simulink model "ElevatorRegen_OptB_L2"  (R2024b)
settings: Solver=FixedStepDiscrete  StartTime=0.0  StopTime=25  FixedStep=Ts_power  RelTol=1e-3
values from neighbouring files (symbols this model uses):
  Cdc = 2.2e-3    (= 0.0022)    [params_elevator.m]
  f_g = 50    [params_elevator.m]
  L_acd = 0.5e-3    (= 0.0005)    [params_elevator.m]
  L_f = L1 + L2    [params_elevator.m]
  Lg = XR*Rg/w_g    [params_elevator.m]
  R_acd = 5e-3    (= 0.005)    [params_elevator.m]
  R_f = 0.005*Z_B    (= 0.0666666666667)    [params_elevator.m]
  Rb_B = Vchop_on^2/P_DC_regen_peak    (= 48.4015424137)    [params_elevator.m]
  Rg = Zg/sqrt(1+XR^2)    [params_elevator.m]
  SIGNE_ISRC = +1    (= 1)    [build_optionB_L2.m]
  Ts_ctrl = 1/fsw    (= 0.0001)    [params_elevator.m]
  Ts_power = Ts_ctrl/2    (= 5e-05)    [params_elevator.m]
  V_LL = 400    [params_elevator.m]
  Vchop_off = 740    [params_elevator.m]
  Vchop_on = 760    [params_elevator.m]
libraries: spsThreePhaseSeriesRLCBranchLib x3, spsControlledVoltageSourceLib x3, spsSeriesRLCBranchLib x2, spsControlledCurrentSourceLib x2, spsThreePhaseVIMeasurementLib x2, spsIdealSwitchLib x1, spsVoltageMeasurementLib x1, spsUniversalBridgeLib x1, spsThreePhaseSourceLib x1, spspowerguiLib x1
settings Model: Creator=Med Amine  LastModifiedBy=Med Amine

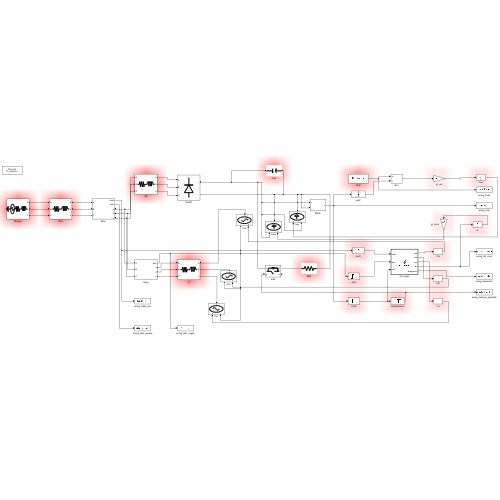
[thumbnail: Simulink's stored preview of the top-level diagram]
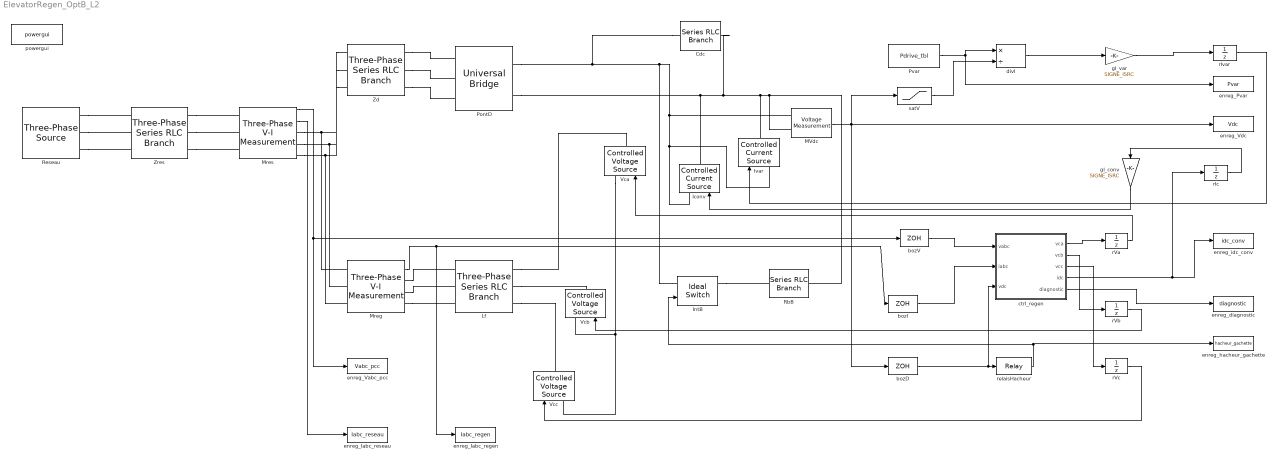
== system ElevatorRegen_OptB_L2 ==
  Cdc : spsSeriesRLCBranchLib/Series RLC Branch  LConnTagsString=__new0  RConnTagsString=__new0  BranchType=C  Resistance=1  Inductance=1e-3  SetiL0=on  InitialCurrent=0  Capacitance=Cdc  Setx0=off  InitialVoltage=Vdc0  Measurements=None
  Iconv : spsControlledCurrentSourceLib/Controlled Current Source  Initialize=on  Source_Type=AC  Amplitude=0  Phase=0  Frequency=0  Measurements=None
  IntB : spsIdealSwitchLib/Ideal Switch  Ron=1e-3  Lon=0  IC=0  Rs=1e6  Cs=inf  Measurements=on
  Ivar : spsControlledCurrentSourceLib/Controlled Current Source  Initialize=on  Source_Type=AC  Amplitude=0  Phase=0  Frequency=0  Measurements=None
  Lf : spsThreePhaseSeriesRLCBranchLib/Three-Phase Series RLC Branch  LConnTagsString=A|B|C  RConnTagsString=A|B|C  BranchType=RL  Resistance=R_f  Inductance=L_f  Capacitance=1e-6  Measurements=None
  MVdc : spsVoltageMeasurementLib/Voltage Measurement  PhasorSimulation=off  OutputType=Complex  PSBequivalent=0
  Mreg : spsThreePhaseVIMeasurementLib/Three-Phase V-I Measurement  VoltageMeasurement=no  SetLabelV=off  LabelV=Vabc  Vpu=off  VpuLL=off  CurrentMeasurement=yes  SetLabelI=off  LabelI=Iabc  Ipu=off  Pbase=100e6  Vbase=500e3  OutputType=Complex  PhasorSimulation=off  PSBequivalent=0
  Mres : spsThreePhaseVIMeasurementLib/Three-Phase V-I Measurement  VoltageMeasurement=phase-to-ground  SetLabelV=off  LabelV=Vabc  Vpu=off  VpuLL=off  CurrentMeasurement=yes  SetLabelI=off  LabelI=Iabc  Ipu=off  Pbase=100e6  Vbase=500e3  OutputType=Complex  PhasorSimulation=off  PSBequivalent=0
  PontD : spsUniversalBridgeLib/Universal Bridge  Arms=3  SnubberResistance=1e5  SnubberCapacitance=inf  Device=Diodes  Ron=1e-3  Lon=0  ForwardVoltages="[  0  0  ]"  ForwardVoltage=0.8  GTOparameters=[ 10e-6 , 20e-6 ]  IGBTparameters=[ 1e-6 , 2e-6 ]  Measurements=None  Measurements_2=None  converterType=Rectifier
  Pvar : FromWorkspace  VariableName=Pdrive_tbl  OutputAfterFinalValue=Setting to zero
  RbB : spsSeriesRLCBranchLib/Series RLC Branch  LConnTagsString=__new0  RConnTagsString=__new0  BranchType=R  Resistance=Rb_B  Inductance=1e-3  SetiL0=off  InitialCurrent=0  Capacitance=1e-6  Setx0=off  InitialVoltage=0  Measurements=None
  Reseau : spsThreePhaseSourceLib/Three-Phase Source  InternalConnection=Yg  VoltagePhases=off  Voltage=V_LL  PhaseAngle=0  Voltage_phases=[25e3 25e3 25e3]/sqrt(3)  PhaseAngles_phases=[0 -120 +120]  Frequency=f_g  NonIdealSource=on  SpecifyImpedance=off  Resistance=0.8929  Inductance=16.58e-3  ShortCircuitLevel=100e6  BaseVoltage=25e3  XRratio=7  BusType=swing  Pref=10e3  Qref=0  Prefabc=[10e3, 10e3, 10e3]  Qrefabc=[0, 0, 0]  Qmin=-inf  Qmax=inf
  Vca : spsControlledVoltageSourceLib/Controlled Voltage Source  Initialize=on  Source_Type=AC  Amplitude=0  Phase=0  Frequency=0  Measurements=None
  Vcb : spsControlledVoltageSourceLib/Controlled Voltage Source  Initialize=on  Source_Type=AC  Amplitude=0  Phase=0  Frequency=0  Measurements=None
  Vcc : spsControlledVoltageSourceLib/Controlled Voltage Source  Initialize=on  Source_Type=AC  Amplitude=0  Phase=0  Frequency=0  Measurements=None
  Zd : spsThreePhaseSeriesRLCBranchLib/Three-Phase Series RLC Branch  LConnTagsString=A|B|C  RConnTagsString=A|B|C  BranchType=RL  Resistance=R_acd  Inductance=L_acd  Capacitance=1e-6  Measurements=None
  Zres : spsThreePhaseSeriesRLCBranchLib/Three-Phase Series RLC Branch  LConnTagsString=A|B|C  RConnTagsString=A|B|C  BranchType=RL  Resistance=Rg  Inductance=Lg  Capacitance=1e-6  Measurements=None
  bozD : ZeroOrderHold  SampleTime=Ts_ctrl
  bozI : ZeroOrderHold  SampleTime=Ts_ctrl
  bozV : ZeroOrderHold  SampleTime=Ts_ctrl
  ctrl_regen : MATLAB Function  TreatAsAtomicUnit=on
  divI : Product  Inputs=*/
  enreg_Iabc_regen : ToWorkspace  VariableName=Iabc_regen  SaveFormat=Timeseries  SampleTime=-1
  enreg_Iabc_reseau : ToWorkspace  VariableName=Iabc_reseau  SaveFormat=Timeseries  SampleTime=-1
  enreg_Pvar : ToWorkspace  VariableName=Pvar  SaveFormat=Timeseries  SampleTime=-1
  enreg_Vabc_pcc : ToWorkspace  VariableName=Vabc_pcc  SaveFormat=Timeseries  SampleTime=-1
  enreg_Vdc : ToWorkspace  VariableName=Vdc  SaveFormat=Timeseries  SampleTime=-1
  enreg_diagnostic : ToWorkspace  VariableName=diagnostic  SaveFormat=Timeseries  SampleTime=-1
  enreg_hacheur_gachette : ToWorkspace  VariableName=hacheur_gachette  SaveFormat=Timeseries  SampleTime=-1
  enreg_idc_conv : ToWorkspace  VariableName=idc_conv  SaveFormat=Timeseries  SampleTime=-1
  gI_conv : Gain  Gain=SIGNE_ISRC
  gI_var : Gain  Gain=SIGNE_ISRC
  powergui : spspowerguiLib/powergui  Priority=1  SimulationMode=Discrete  SampleTime=Ts_power  frequency=60  Iterations=50  frequencyindice=60  Pbase=100e6  ErrMax=1e-4  UnitsV=kV  UnitsW=MW  buscounter=0  FunctionMessages=off  echomessages=off  EnableUseOfTLC=off  CurrentSourceSwitches=off  DisableSnubberDevices=off  DisableRonSwitches=off  DisableVfSwitches=off  DisplayEquations=off  AutomaticDiscreteSolvers=off  SolverType=Tustin/Backward Euler (TBE)  Interpol=off  ExternalGateDelay=off  methode=off  Ts=100  x0status=blocks  SPID=on  SwTol=0  HookPort=off  NonlinearTolerance=1e-4  nMaxIteration=100  ContinueOnMaxIteration=off  RestoreLinks=warning  ResistiveCurrentMeasurement=off  Frange=[0:2:500]  Ylog=off  Xlog=on  ShowGrid=off  save=off  variable=ZData  structure=0  ZoomFFT=off  StartTime=0.0  cycles=1  DisplayStyle=1  fundamental=60  FreqAxis=off  MaxFrequency=1000  frequencyindicesteady=1  RmsSteady=1  display=off
  rIc : UnitDelay  SampleTime=Ts_ctrl  HasFrameUpgradeWarning=on
  rIvar : UnitDelay  SampleTime=Ts_power  HasFrameUpgradeWarning=on
  rVa : UnitDelay  SampleTime=Ts_ctrl  HasFrameUpgradeWarning=on
  rVb : UnitDelay  SampleTime=Ts_ctrl  HasFrameUpgradeWarning=on
  rVc : UnitDelay  SampleTime=Ts_ctrl  HasFrameUpgradeWarning=on
  relaisHacheur : Relay  OnSwitchValue=Vchop_on  OffSwitchValue=Vchop_off
  satV : Saturate  UpperLimit=2000  LowerLimit=100
  wires:
  MVdc/1 -> enreg_Vdc/1, bozD/1, satV/1
  Pvar/1 -> enreg_Pvar/1, divI/1
  Mres/1 -> bozV/1, enreg_Vabc_pcc/1
  Mres/2 -> enreg_Iabc_reseau/1
  Mreg/1 -> bozI/1, enreg_Iabc_regen/1
  ctrl_regen/4(idc) -> enreg_idc_conv/1, rIc/1
  ctrl_regen/5(diagnostic) -> enreg_diagnostic/1
  relaisHacheur/1 -> enreg_hacheur_gachette/1, IntB/1
  bozV/1 -> ctrl_regen/1(vabc)
  bozI/1 -> ctrl_regen/2(iabc)
  bozD/1 -> ctrl_regen/3(vdc), relaisHacheur/1
  rIc/1 -> gI_conv/1
  gI_conv/1 -> Iconv/1
  satV/1 -> divI/2
  divI/1 -> gI_var/1
  gI_var/1 -> rIvar/1
  rIvar/1 -> Ivar/1
  ctrl_regen/1(vca) -> rVa/1
  rVa/1 -> Vca/1
  ctrl_regen/2(vcb) -> rVb/1
  rVb/1 -> Vcb/1
  ctrl_regen/3(vcc) -> rVc/1
  rVc/1 -> Vcc/1
  connections:
  Reseau/RConn1 -- Zres/LConn1
  Zres/RConn1 -- Mres/LConn1
  Zd/LConn1 -- Mres/RConn1 -- Mreg/LConn1
  Zd/RConn1 -- PontD/LConn1
  Mreg/RConn1 -- Lf/LConn1
  Lf/RConn1 -- Vca/RConn1
  Reseau/RConn2 -- Zres/LConn2
  Zres/RConn2 -- Mres/LConn2
  Zd/LConn2 -- Mres/RConn2 -- Mreg/LConn2
  Zd/RConn2 -- PontD/LConn2
  Mreg/RConn2 -- Lf/LConn2
  Lf/RConn2 -- Vcb/RConn1
  Reseau/RConn3 -- Zres/LConn3
  Zres/RConn3 -- Mres/LConn3
  Zd/LConn3 -- Mres/RConn3 -- Mreg/LConn3
  Zd/RConn3 -- PontD/LConn3
  Mreg/RConn3 -- Lf/LConn3
  Lf/RConn3 -- Vcc/RConn1
  Vca/LConn1 -- Vcb/LConn1 -- Vcc/LConn1
  Cdc/LConn1 -- PontD/RConn1 -- Ivar/LConn1 -- Iconv/LConn1 -- MVdc/LConn1 -- IntB/LConn1
  Cdc/RConn1 -- PontD/RConn2 -- Iconv/RConn1 -- Ivar/RConn1 -- RbB/RConn1 -- MVdc/LConn2
  IntB/RConn1 -- RbB/LConn1

== matlab function ElevatorRegen_OptB_L2/ctrl_regen ==
  data: vabc input; vca output; iabc input; vdc input; vcb output; vcc output; idc output; diagnostic output
function [vca, vcb, vcc, idc, diagnostic] = ctrl_regen(vabc, iabc, vdc)
% Commande de regeneration seule, option B : boucle a verrouillage de phase (PLL) en repere synchrone,
% boucle de tension DC unidirectionnelle, boucle de courant dq.
persistent th wint xid xiq xv
if isempty(th)
    th = 0; wint = 0; xid = 0; xiq = 0; xv = 0;
end
Ts = 0.0001; w0 = 314.159265; Vpk = 326.598632; Lf = 0.00265850868; SGN = 1;
kpi = 8.8616956; kii = 222.222222; kpv = 0.778119927; kiv = 103.712872; kpp = 444.288294; kip = 98696.044;
Vreg = 650; Idmax = 26.7950793;
va = vabc(1); vb = vabc(2); vc = vabc(3);
ia = -iabc(1); ib = -iabc(2); ic = -iabc(3);   % courant INJECTE dans le reseau
% Clarke (invariant en amplitude) et Park
va_al = (2/3)*(va - 0.5*vb - 0.5*vc);  va_be = (vb - vc)/sqrt(3);
ia_al = (2/3)*(ia - 0.5*ib - 0.5*ic);  ia_be = (ib - ic)/sqrt(3);
cs = cos(th); sn = sin(th);
vd =  va_al*cs + va_be*sn;   vq = -va_al*sn + va_be*cs;
id =  ia_al*cs + ia_be*sn;   iq = -ia_al*sn + ia_be*cs;
% PLL (PI sur vq normalise)
e_pll = vq/Vpk;
wint  = wint + kip*Ts*e_pll;
w     = w0 + kpp*e_pll + wint;
th_n  = th + w*Ts;  th_n = th_n - 2*pi*floor(th_n/(2*pi));
% Boucle de tension DC : sortie limitee a [0, Idmax] -> le convertisseur ne soutire jamais de puissance
vlim   = max(vdc,100)/sqrt(3);
ev     = vdc - Vreg;
idr_u  = kpv*ev + xv;
idref  = min(max(idr_u,0), Idmax);
if ~(idr_u >= Idmax && ev > 0)
    xv = min(max(xv + kiv*Ts*ev, 0), Idmax);
end
% Boucle de courant dq avec decouplage croise et anticipation de la tension reseau
eid = idref - id;  eiq = 0 - iq;
xid = min(max(xid + kii*Ts*eid, -vlim), vlim);
xiq = min(max(xiq + kii*Ts*eiq, -vlim), vlim);
vcd = vd - w*Lf*iq + kpi*eid + xid;
vcq = vq + w*Lf*id + kpi*eiq + xiq;
vm = hypot(vcd, vcq);
if vm > vlim, vcd = vcd*vlim/vm; vcq = vcq*vlim/vm; end
% retour en abc
v_al = vcd*cs - vcq*sn;  v_be = vcd*sn + vcq*cs;
va_c = v_al;  vb_c = -0.5*v_al + (sqrt(3)/2)*v_be;  vc_c = -0.5*v_al - (sqrt(3)/2)*v_be;
% cote DC moyen : bilan de puissance instantane (sans pertes au niveau L2)
p   = va_c*ia + vb_c*ib + vc_c*ic;      % puissance fournie au reseau
idc = p/max(vdc,100);                   % courant preleve sur le bus DC
vca = SGN*va_c; vcb = SGN*vb_c; vcc = SGN*vc_c;
diagnostic = [id; iq; idref; w/(2*pi); vd];
th = th_n;
